simulink model "ADCSSimulator"  (R2024a)
settings: Solver=ode4  StartTime=0.0  StopTime=600  FixedStep=0.01  MaxStep=0.1  RelTol=1e-3  AbsTol=1e-3
values from neighbouring files (symbols this model uses):
  ActuatorAllocationMatrix = ActuatorPhysicalMatrix' * inv(ActuatorPhysicalMatrix * ActuatorPhysicalMatrix')    [set_Init.m]
  ActuatorPhysicalMatrix = [1, 0, 0, 0 ... (first row only)    [set_Init.m]
  albedo_irradiance = 300    [set_Init.m]
  b = 0    [set_Init.m]
  Cd = 2.2    [set_Init.m]
  h_bias = [0; 0; 0]    [set_Init.m]
  J = 4.0e-3 / 628    (= 6.36942675159e-06)    [set_Init.m]
  k_Bdot = ((4 * pi * 0.5236 * 0.0055) / (5677.2 * (4.5e-5)^2))    (= 3147.8423197)    [set_Init.m]
  K_E = K_T    (= 0.0022)    [set_Init.m]
  K_T = 0.0022    [set_Init.m]
  P0 = blkdiag(P0_att, P0_bias)    [set_Init.m]
  P0_att = eye(3) * initial_variance_rad2    [set_Init.m]
  PowerVoltageBus_01 = 3.3    [set_Init.m]
  PowerVoltageBus_02 = 3.3    [set_Init.m]
  PowerVoltageBus_03 = 3.3    [set_Init.m]
  PowerVoltageBus_04 = 3.3    [set_Init.m]
  PowerVoltageBus_05 = 3.3    [set_Init.m]
  PowerVoltageBus_06 = 3.3    [set_Init.m]
  PowerVoltageBus_07 = 3.3    [set_Init.m]
  PowerVoltageBus_08 = 3.3    [set_Init.m]
  PowerVoltageBus_09 = 3.3    [set_Init.m]
  PowerVoltageBus_10 = 3.3    [set_Init.m]
  PowerVoltageBus_11 = 3.3    [set_Init.m]
  PowerVoltageBus_12 = 0.0    (= 0)    [set_Init.m]
  PowerVoltageBus_13 = 0.0    (= 0)    [set_Init.m]
  PowerVoltageBus_14 = 0.0    (= 0)    [set_Init.m]
  PowerVoltageBus_15 = 0.0    (= 0)    [set_Init.m]
  R = 2.0    (= 2)    [set_Init.m]
  ressidual_m = [3e-4; -2e-4; 1e-4]    [set_Init.m]
  solar_irradiance = 1361    [set_Init.m]
  surface_areas = [A_xy, A_yz, A_xz, A_xy, A_yz, A_xz]    [set_Init.m]
  surface_normals_body = [eye(3) -eye(3)]    [set_Init.m]
  surface_positions_body = [       hx,   0,   0 ... (first row only)    [set_Init.m]
  surface_reflectivities = [0.9 0.8 0.9 0.9 0.9 0.9]    [set_Init.m]
  Switch_01 = 1    [set_Init.m]
  Switch_02 = 1    [set_Init.m]
  Switch_03 = 1    [set_Init.m]
  Switch_04 = 1    [set_Init.m]
  Switch_05 = 1    [set_Init.m]
  Switch_06 = 1    [set_Init.m]
  Switch_07 = 1    [set_Init.m]
  Switch_08 = 1    [set_Init.m]
  Switch_09 = 1    [set_Init.m]
  Switch_10 = 1    [set_Init.m]
  Switch_11 = 1    [set_Init.m]
  Switch_12 = 0    [set_Init.m]
  Switch_13 = 0    [set_Init.m]
  Switch_14 = 0    [set_Init.m]
  Switch_15 = 0    [set_Init.m]
  visSampleTime = 0.1    [set_Init.m]
undefined symbols (not defined in the file or in its folder): attitude, Controller, epoch, IAU, juliandate, Kd, km, Kp, m, rad, s, satellite, SGP4_parameters, simulator, UKF_parameters, WMM2020
libraries: sharedtransform x27, aerolibutil x22, aerolibconvert2 x18, simulink_extras x16, matrix_library x6, aerolibtransform2 x4, vrlib x2, aerolibgravity2 x2, aerolibobsolete x1, aerolibattitudesys x1, simulink x1
(part 7 of 8)

== matlab function ADCSSimulator/ADCS/ADCS Software/Onboard Reference Frames Transformations Manager1/Ensure Quaternion Continuity1/Ensure Quaternion Continuity ==
  data: q_new input; q_out output; q_prev input
function q_out = quaternion_continuity(q_new, q_prev)
%%%%%%%%%%%%%%%%%%%%%%%%%%%%%%%%%%%%%%%%%%%%%%%%%%%%%%%%%%%%%%%%%%%%%%%%
%   QUATERNION_CONTINUITY Ensures continuous quaternion output.
%
%   q_out = ensure_quaternion_continuity(q_new, q_prev) selects between
%   q_new and -q_new to ensure the shortest rotational path from q_prev,
%   preventing sign-flipping discontinuities in simulations.
%
%   Inputs:
%       q_new   - 4x1 newly calculated quaternion. Can be in either
%                 scalar-first or scalar-last format.
%       q_prev  - 4x1 quaternion from the previous time step. Must be in
%                 the same format as q_new.
%
%   Output:
%       q_out   - The 4x1 quaternion (either q_new or -q_new) that is
%                 mathematically closer to q_prev.
%%%%%%%%%%%%%%%%%%%%%%%%%%%%%%%%%%%%%%%%%%%%%%%%%%%%%%%%%%%%%%%%%%%%%%%%

    % 1. Input Validation (optional for Simulink if types are enforced)
    % coder.extrinsic('error'); % Uncomment if you need error checking
    % if ~isequal(size(q_new), [4,1]) || ~isequal(size(q_prev), [4,1])
    %     error('Input quaternions must be 4x1 column vectors.');
    % end

    % 2. Calculate the Euclidean distance (norm) to both possible rotations
    % The quaternions q and -q represent the same physical rotation. We want
    % to choose the one that is numerically closer to the previous state to
    % avoid a "jump" in the data when plotted.
    dist_to_positive_q = norm(q_new - q_prev);
    dist_to_negative_q = norm(-q_new - q_prev);

    % 3. Select the quaternion on the shortest path
    if dist_to_negative_q < dist_to_positive_q
        q_out = -q_new;
    else
        q_out = q_new;
    end
end

== matlab function ADCSSimulator/ADCS/ADCS Software/Onboard Reference Frames Transformations Manager1/Ensure Quaternion Continuity2/Ensure Quaternion Continuity ==
  data: q_new input; q_out output; q_prev input
function q_out = quaternion_continuity(q_new, q_prev)
%%%%%%%%%%%%%%%%%%%%%%%%%%%%%%%%%%%%%%%%%%%%%%%%%%%%%%%%%%%%%%%%%%%%%%%%
%   QUATERNION_CONTINUITY Ensures continuous quaternion output.
%
%   q_out = ensure_quaternion_continuity(q_new, q_prev) selects between
%   q_new and -q_new to ensure the shortest rotational path from q_prev,
%   preventing sign-flipping discontinuities in simulations.
%
%   Inputs:
%       q_new   - 4x1 newly calculated quaternion. Can be in either
%                 scalar-first or scalar-last format.
%       q_prev  - 4x1 quaternion from the previous time step. Must be in
%                 the same format as q_new.
%
%   Output:
%       q_out   - The 4x1 quaternion (either q_new or -q_new) that is
%                 mathematically closer to q_prev.
%%%%%%%%%%%%%%%%%%%%%%%%%%%%%%%%%%%%%%%%%%%%%%%%%%%%%%%%%%%%%%%%%%%%%%%%

    % 1. Input Validation (optional for Simulink if types are enforced)
    % coder.extrinsic('error'); % Uncomment if you need error checking
    % if ~isequal(size(q_new), [4,1]) || ~isequal(size(q_prev), [4,1])
    %     error('Input quaternions must be 4x1 column vectors.');
    % end

    % 2. Calculate the Euclidean distance (norm) to both possible rotations
    % The quaternions q and -q represent the same physical rotation. We want
    % to choose the one that is numerically closer to the previous state to
    % avoid a "jump" in the data when plotted.
    dist_to_positive_q = norm(q_new - q_prev);
    dist_to_negative_q = norm(-q_new - q_prev);

    % 3. Select the quaternion on the shortest path
    if dist_to_negative_q < dist_to_positive_q
        q_out = -q_new;
    else
        q_out = q_new;
    end
end

== matlab function ADCSSimulator/ADCS/ADCS Software/Onboard Reference Frames Transformations Manager1/Ensure Quaternion Continuity3/Ensure Quaternion Continuity ==
  data: q_new input; q_out output; q_prev input
function q_out = quaternion_continuity(q_new, q_prev)
%%%%%%%%%%%%%%%%%%%%%%%%%%%%%%%%%%%%%%%%%%%%%%%%%%%%%%%%%%%%%%%%%%%%%%%%
%   QUATERNION_CONTINUITY Ensures continuous quaternion output.
%
%   q_out = ensure_quaternion_continuity(q_new, q_prev) selects between
%   q_new and -q_new to ensure the shortest rotational path from q_prev,
%   preventing sign-flipping discontinuities in simulations.
%
%   Inputs:
%       q_new   - 4x1 newly calculated quaternion. Can be in either
%                 scalar-first or scalar-last format.
%       q_prev  - 4x1 quaternion from the previous time step. Must be in
%                 the same format as q_new.
%
%   Output:
%       q_out   - The 4x1 quaternion (either q_new or -q_new) that is
%                 mathematically closer to q_prev.
%%%%%%%%%%%%%%%%%%%%%%%%%%%%%%%%%%%%%%%%%%%%%%%%%%%%%%%%%%%%%%%%%%%%%%%%

    % 1. Input Validation (optional for Simulink if types are enforced)
    % coder.extrinsic('error'); % Uncomment if you need error checking
    % if ~isequal(size(q_new), [4,1]) || ~isequal(size(q_prev), [4,1])
    %     error('Input quaternions must be 4x1 column vectors.');
    % end

    % 2. Calculate the Euclidean distance (norm) to both possible rotations
    % The quaternions q and -q represent the same physical rotation. We want
    % to choose the one that is numerically closer to the previous state to
    % avoid a "jump" in the data when plotted.
    dist_to_positive_q = norm(q_new - q_prev);
    dist_to_negative_q = norm(-q_new - q_prev);

    % 3. Select the quaternion on the shortest path
    if dist_to_negative_q < dist_to_positive_q
        q_out = -q_new;
    else
        q_out = q_new;
    end
end

== matlab function ADCSSimulator/ADCS/ADCS Software/Onboard Reference Frames Transformations Manager1/Ensure Quaternion Continuity4/Ensure Quaternion Continuity ==
  data: q_new input; q_out output; q_prev input
function q_out = quaternion_continuity(q_new, q_prev)
%%%%%%%%%%%%%%%%%%%%%%%%%%%%%%%%%%%%%%%%%%%%%%%%%%%%%%%%%%%%%%%%%%%%%%%%
%   QUATERNION_CONTINUITY Ensures continuous quaternion output.
%
%   q_out = ensure_quaternion_continuity(q_new, q_prev) selects between
%   q_new and -q_new to ensure the shortest rotational path from q_prev,
%   preventing sign-flipping discontinuities in simulations.
%
%   Inputs:
%       q_new   - 4x1 newly calculated quaternion. Can be in either
%                 scalar-first or scalar-last format.
%       q_prev  - 4x1 quaternion from the previous time step. Must be in
%                 the same format as q_new.
%
%   Output:
%       q_out   - The 4x1 quaternion (either q_new or -q_new) that is
%                 mathematically closer to q_prev.
%%%%%%%%%%%%%%%%%%%%%%%%%%%%%%%%%%%%%%%%%%%%%%%%%%%%%%%%%%%%%%%%%%%%%%%%

    % 1. Input Validation (optional for Simulink if types are enforced)
    % coder.extrinsic('error'); % Uncomment if you need error checking
    % if ~isequal(size(q_new), [4,1]) || ~isequal(size(q_prev), [4,1])
    %     error('Input quaternions must be 4x1 column vectors.');
    % end

    % 2. Calculate the Euclidean distance (norm) to both possible rotations
    % The quaternions q and -q represent the same physical rotation. We want
    % to choose the one that is numerically closer to the previous state to
    % avoid a "jump" in the data when plotted.
    dist_to_positive_q = norm(q_new - q_prev);
    dist_to_negative_q = norm(-q_new - q_prev);

    % 3. Select the quaternion on the shortest path
    if dist_to_negative_q < dist_to_positive_q
        q_out = -q_new;
    else
        q_out = q_new;
    end
end

== matlab function ADCSSimulator/ADCS/ADCS Software/Onboard Reference Frames Transformations Manager1/Ensure Quaternion Continuity5/Ensure Quaternion Continuity ==
  data: q_new input; q_out output; q_prev input
function q_out = quaternion_continuity(q_new, q_prev)
%%%%%%%%%%%%%%%%%%%%%%%%%%%%%%%%%%%%%%%%%%%%%%%%%%%%%%%%%%%%%%%%%%%%%%%%
%   QUATERNION_CONTINUITY Ensures continuous quaternion output.
%
%   q_out = ensure_quaternion_continuity(q_new, q_prev) selects between
%   q_new and -q_new to ensure the shortest rotational path from q_prev,
%   preventing sign-flipping discontinuities in simulations.
%
%   Inputs:
%       q_new   - 4x1 newly calculated quaternion. Can be in either
%                 scalar-first or scalar-last format.
%       q_prev  - 4x1 quaternion from the previous time step. Must be in
%                 the same format as q_new.
%
%   Output:
%       q_out   - The 4x1 quaternion (either q_new or -q_new) that is
%                 mathematically closer to q_prev.
%%%%%%%%%%%%%%%%%%%%%%%%%%%%%%%%%%%%%%%%%%%%%%%%%%%%%%%%%%%%%%%%%%%%%%%%

    % 1. Input Validation (optional for Simulink if types are enforced)
    % coder.extrinsic('error'); % Uncomment if you need error checking
    % if ~isequal(size(q_new), [4,1]) || ~isequal(size(q_prev), [4,1])
    %     error('Input quaternions must be 4x1 column vectors.');
    % end

    % 2. Calculate the Euclidean distance (norm) to both possible rotations
    % The quaternions q and -q represent the same physical rotation. We want
    % to choose the one that is numerically closer to the previous state to
    % avoid a "jump" in the data when plotted.
    dist_to_positive_q = norm(q_new - q_prev);
    dist_to_negative_q = norm(-q_new - q_prev);

    % 3. Select the quaternion on the shortest path
    if dist_to_negative_q < dist_to_positive_q
        q_out = -q_new;
    else
        q_out = q_new;
    end
end

== matlab function ADCSSimulator/ADCS/ADCS Software/Onboard Reference Frames Transformations Manager1/MATLAB Function ==
  data: r input; SemiMajorAxis output; v input; mu input; Eccentricity output; Inclination output; RightAscension output; ArgumentOfPerigee output; TrueAnomaly output; TrueLongitude output; ArgumentOfLatitude output; LongitudeOfPeriapsis output; SemilatusRectum output; OrbOmega output
%----------------------- Begin Code Sequence -----------------------------%
% Purpose:                                                                %
% Convert a given set of state vectors in ECI reference frame to orbital  %
% elements.                                                               %
%-------------------------------------------------------------------------%
%                                                                         %
% Inputs:                                                                 %
%--------                                                                  
%r_ECI                  [3 x N]                         Position Vector in
%                                                       ECI coordinate
%                                                       frame of reference
%
%v_ECI                  [3 x N]                         Velocity vector in
%                                                       ECI coordinate
%                                                       frame of reference
%
%mu                     double                          Gravitational Constant
%                                                       Defaults to Earth if
%                                                       not specified
% Outputs:
%---------                                                                %
%a                      [1 x N]                         Semi-Major Axis
%                                                       (m)
%
%eMag                   [1 x N]                         Eccentricity
%                                                       (unitless)
%
%i                      [1 x N]                         inclination
%                                                       (rad)
%
%O                      [1 x N]                         Right Ascention of
%                                                       the ascending node
%                                                       (rad)
%
%o                      [1 x N]                         Argument of perigee
%                                                       (rad)
%
%M                      [1 x N]                         Mean Anomaly
%                                                       (rad)
%
%truLon                 [1 x N]                         True Longitude
%                                                       (rad)
%
%argLat                 [1 x N]                         Argument of Latitude
%                                                       (rad)
%
%lonPer                 [1 x N]                         Longitude of Periapse
%                                                       (rad)
%
%p                      [1 x N]                         Semilatus Rectum
%                                                       (m)
%
%OrbOmega                                               Orbital Frame
%                                                       angular velocity
%                                                       (rad)
% References:
%-------------
%Vallado,D. Fundamentals of Astrodynamics and Applications. 2007.
%
% Function Dependencies:
%------------------
%None
%------------------------------------------------------------------       %
% Programed by Darin Koblick  03-04-2012                                  %
% modified by A.H.Khodabakhsh 10-01-2021                                  %
% Updated to address circular equatorial orbits       12/12/2013          %
%------------------------------------------------------------------       %
function [SemiMajorAxis,Eccentricity,Inclination,RightAscension,ArgumentOfPerigee,TrueAnomaly,...
          TrueLongitude,ArgumentOfLatitude,LongitudeOfPeriapsis,SemilatusRectum,OrbOmega] = ...
          StateVector2KeplerianOrbitalElemets(r,v,mu)
% if ~exist('mu','var');  t = getConst(); mu = t.Earth.Mu; end
%Specific angular momentum
h = cross(r,v);
n = cross(repmat([0;0;1],[1,size(r,2)]),h); nMag = sqrt(sum(n.^2,1));
vMag = sqrt(sum(v.^2,1)); 
rMag = sqrt(sum(r.^2,1)); 
hMag = sqrt(sum(h.^2,1));
e = (1./mu).*(bsxfun(@times,(vMag.^2 - mu./rMag),r) - bsxfun(@times,dot(r,v),v)); 
Eccentricity = sqrt(sum(e.^2,1));
zeta = (vMag.^2)./2 - mu./rMag;
%Special Procedure when we have a parabolic orbit
idx = Eccentricity ~= 1;
SemiMajorAxis = zeros(size(Eccentricity));
SemilatusRectum = zeros(size(Eccentricity));
if any(idx)
    SemiMajorAxis(idx) = -mu./(2.*zeta(idx)); 
    SemilatusRectum(idx) = SemiMajorAxis(idx).*(1-Eccentricity(idx).^2); 
else
    SemiMajorAxis(idx) = Inf; 
    SemilatusRectum(idx) = (hMag(idx).^2)./mu; 
end
%Compute the angles
Inclination             = acos(double(single(   h(3,:)./hMag)                   )); 
RightAscension          = acos(double(single(   n(1,:)./nMag)                   ));
ArgumentOfPerigee       = acos(double(single(   dot(n,e)./(nMag.*Eccentricity)) ));
TrueAnomaly             = acos(double(single(   dot(e,r)./(Eccentricity.*rMag)) ));
LongitudeOfPeriapsis    = acos(double(single(   e(1,:)./Eccentricity)           ));
ArgumentOfLatitude      = acos(double(single(   dot(n,r)./(nMag.*rMag))         ));
TrueLongitude           = acos(double(single(   r(1,:)./rMag)                   ));
%Account for those cases where satellite is in circular orbit
         RightAscension   (  n(1,:) == 0) = 0;
       ArgumentOfPerigee  (dot(n,e) == 0) = 0;
      LongitudeOfPeriapsis(  e(1,:) == 0) = 0;
          TrueAnomaly     (dot(e,r) == 0) = 0;
       ArgumentOfLatitude (dot(n,r) == 0) = 0;
%Apply Quadrant Checks to All Determined Angles
idx = n(2,:) < 0; if any(idx),  RightAscension(idx) = 2*pi - RightAscension(idx);  end;
idx = e(3,:) < 0; if any(idx), ArgumentOfPerigee(idx) = 2*pi - ArgumentOfPerigee(idx); end;
idx = dot(r,v) < 0; if any(idx), TrueAnomaly(idx) = 2*pi - TrueAnomaly(idx); end;
idx = e(2,:) < 0; if any(idx), LongitudeOfPeriapsis(idx) = 2*pi-LongitudeOfPeriapsis(idx);  end;
idx = r(3,:) < 0; if any(idx), ArgumentOfLatitude(idx) = 2*pi - ArgumentOfLatitude(idx); end;
idx = r(2,:) < 0; if any(idx), TrueLongitude(idx) = 2*pi - TrueLongitude(idx); end;

rv = zeros(3,1);
rv(:)=cross(r,v); norm_r = norm(r);
OrbOmega = [0;
            dot(v,cross(r./norm_r,rv./norm(rv)))/norm_r;
            0];

% % convert radians to degrees
% r2d = @(x) x.*(180./pi);
% Inclination          = r2d(Inclination         );
% RightAscension       = r2d(RightAscension      );
% ArgumentOfPerigee    = r2d(ArgumentOfPerigee   );
% TrueAnomaly          = r2d(TrueAnomaly         );
% TrueLongitude        = r2d(TrueLongitude       );
% ArgumentOfLatitude   = r2d(ArgumentOfLatitude  );
% LongitudeOfPeriapsis = r2d(LongitudeOfPeriapsis);
% OrbOmega             = r2d(OrbOmega            );
end

== matlab function ADCSSimulator/ADCS/ADCS Software/Attitude Determination/Attitude Estimation Algorithm (MEKF)/Ensure Quaternion Continuity/Ensure Quaternion Continuity ==
  data: q_new input; q_out output; q_prev input
function q_out = quaternion_continuity(q_new, q_prev)
%%%%%%%%%%%%%%%%%%%%%%%%%%%%%%%%%%%%%%%%%%%%%%%%%%%%%%%%%%%%%%%%%%%%%%%%
%   QUATERNION_CONTINUITY Ensures continuous quaternion output.
%
%   q_out = ensure_quaternion_continuity(q_new, q_prev) selects between
%   q_new and -q_new to ensure the shortest rotational path from q_prev,
%   preventing sign-flipping discontinuities in simulations.
%
%   Inputs:
%       q_new   - 4x1 newly calculated quaternion. Can be in either
%                 scalar-first or scalar-last format.
%       q_prev  - 4x1 quaternion from the previous time step. Must be in
%                 the same format as q_new.
%
%   Output:
%       q_out   - The 4x1 quaternion (either q_new or -q_new) that is
%                 mathematically closer to q_prev.
%%%%%%%%%%%%%%%%%%%%%%%%%%%%%%%%%%%%%%%%%%%%%%%%%%%%%%%%%%%%%%%%%%%%%%%%

    % 1. Input Validation (optional for Simulink if types are enforced)
    % coder.extrinsic('error'); % Uncomment if you need error checking
    % if ~isequal(size(q_new), [4,1]) || ~isequal(size(q_prev), [4,1])
    %     error('Input quaternions must be 4x1 column vectors.');
    % end

    % 2. Calculate the Euclidean distance (norm) to both possible rotations
    % The quaternions q and -q represent the same physical rotation. We want
    % to choose the one that is numerically closer to the previous state to
    % avoid a "jump" in the data when plotted.
    dist_to_positive_q = norm(q_new - q_prev);
    dist_to_negative_q = norm(-q_new - q_prev);

    % 3. Select the quaternion on the shortest path
    if dist_to_negative_q < dist_to_positive_q
        q_out = -q_new;
    else
        q_out = q_new;
    end
end

== matlab function ADCSSimulator/ADCS/ADCS Software/Attitude Determination/Attitude Estimation Algorithm (MEKF)/MATLAB Function ==
  data: q_est output; b_est output; P_est output; q_feedback input; b_feedback input; P_feedback input; gyro_meas input; b_sun input; b_mag input; r_sun input; r_mag input; dt input; Q_v input; Q_u input; R_sun input; R_mag input; time input; q_quest input
function [q_est, b_est, P_est] = mekf_quest_reset( ...
    q_feedback, b_feedback, P_feedback, ...
    gyro_meas, b_sun, b_mag, r_sun, r_mag, ...
    dt, Q_v, Q_u, R_sun, R_mag, ...
    time, q_quest)
% MEKF_QUEST_RESET (6-State, Batch Update, One-Time Init)
%
% This function implements a 6-state MEKF with a one-time state reset
% using an external QUEST solution at a specified time.
%
% QUATERNION CONVENTION
% This function uses the standard Hamilton convention: q = [w; x; y; z].

% =========================================================================
% 0) INITIALIZATION & STATE MANAGEMENT
% =========================================================================
QUEST_INIT_TIME = 3.0; % The time to perform the reset

if isempty(P_feedback) || norm(P_feedback) == 0
    q_minus = [1; 0; 0; 0];
    b_minus = [0; 0; 0];
    P_att_initial = eye(3) * (pi^2);
    P_bias_initial = eye(3) * (1e-4);
    P_minus = blkdiag(P_att_initial, P_bias_initial);
else
    q_minus = q_feedback;
    b_minus = b_feedback;
    P_minus = P_feedback;
end

% --- One-Time QUEST Initialization ---
if abs(time - QUEST_INIT_TIME) < (dt / 2) && ~any(isnan(q_quest))
    % ACTION: Overwrite attitude with the QUEST solution
    q_minus = q_quest;
    
    % ACTION: Create a new covariance matrix for the attitude part
    % This is a tuning parameter: our assumed uncertainty after a QUEST reset.
    QUEST_RESET_STD_DEV_DEG = 1.0; % e.g., Assume QUEST is accurate to 1 degree
    QUEST_RESET_STD_DEV_RAD = QUEST_RESET_STD_DEV_DEG * (pi/180);
    P_att_after_quest = eye(3) * QUEST_RESET_STD_DEV_RAD^2;
    
    % Keep the filter's current estimate of the bias covariance
    P_bias_current = P_minus(4:6, 4:6);
    
    % Combine to form the new 6x6 covariance
    P_minus = blkdiag(P_att_after_quest, P_bias_current);
end
q_minus = q_minus / norm(q_minus);

% =========================================================================
% 1) PREDICTION (PROPAGATION)
% =========================================================================
omega = gyro_meas - b_minus;

theta_vec = omega * dt;
phi = norm(theta_vec);
if phi > 1e-9
    axis = theta_vec / phi;
    q_delta = [cos(phi / 2); sin(phi / 2) * axis];
else
    q_delta = [1; 0; 0; 0];
end
q_propagated = quat_mult(q_minus, q_delta);
q_propagated = q_propagated / norm(q_propagated);

skew_omega = cross_matrix(omega);
F = [-skew_omega, -eye(3); zeros(3,3), zeros(3,3)];
Phi = expm(F * dt);
Qd = blkdiag(Q_v, Q_u) * dt;
P_propagated = Phi * P_minus * Phi' + Qd;
P_propagated = 0.5 * (P_propagated + P_propagated');

% =========================================================================
% 2) BATCH MEASUREMENT UPDATE (ROBUST PRE-ALLOCATION VERSION)
% =========================================================================
q_est = q_propagated;
b_est = b_minus;
P_est = P_propagated;

is_sun_available = ~any(isnan(b_sun));
is_mag_available = ~any(isnan(b_mag));

% Proceed only if there is at least one valid measurement
if is_sun_available || is_mag_available
    A = quat_to_dcm(q_propagated);

    % 1. Determine size and pre-allocate matrices
    if is_sun_available && is_mag_available
        meas_size = 6;
    else
        meas_size = 3;
    end
    z = zeros(meas_size, 1);
    h = zeros(meas_size, 1);
    H = zeros(meas_size, 6);
    R = zeros(meas_size, meas_size);
    
    % 2. Fill the matrices based on available sensors
    if is_sun_available && is_mag_available
        % Case 1: Both sensors
        z = [b_sun; b_mag];
        h_sun = A * r_sun;
        h_mag = A * r_mag;
        h = [h_sun; h_mag];
        H_sun = [cross_matrix(h_sun), zeros(3,3)];
        H_mag = [cross_matrix(h_mag), zeros(3,3)];
        H = [H_sun; H_mag];
        R = blkdiag(R_sun, R_mag);
        
    elseif is_sun_available % Case 2: Sun only
        z = b_sun;
        h = A * r_sun;
        H = [cross_matrix(h), zeros(3,3)];
        R = R_sun;

    else % Case 3: Mag only (is_mag_available must be true)
        z = b_mag;
        h = A * r_mag;
        H = [cross_matrix(h), zeros(3,3)];
        R = R_mag;
    end
    
    % 3. Perform the Kalman Update
    % This code now runs safely with guaranteed, fully-defined matrices.
    y = z - h;
    S = H * P_propagated * H' + R;
    K = (P_propagated * H') / S;
    
    delta_x = K * y;
    delta_a = delta_x(1:3);
    delta_b = delta_x(4:6);

    delta_q = [1; 0.5 * delta_a];
    delta_q = delta_q / norm(delta_q);
    
    q_est = quat_mult(q_propagated, delta_q);
    b_est = b_minus + delta_b;

    IKH = eye(6) - K * H;
    P_est = IKH * P_propagated * IKH' + K*R*K';
    P_est = 0.5 * (P_est + P_est');
end

% =========================================================================
% HELPER FUNCTIONS
% =========================================================================
function C = cross_matrix(v)
    C = [  0   -v(3)  v(2); v(3)   0   -v(1); -v(2)  v(1)   0  ];
end

function r = quat_mult(q1, q2)
    w1 = q1(1); v1 = q1(2:4);
    w2 = q2(1); v2 = q2(2:4);
    w = w1*w2 - dot(v1, v2);
    v = w1*v2 + w2*v1 + cross(v1, v2);
    r = [w; v];
end

function A = quat_to_dcm(q)
    w = q(1); v = q(2:4);
    skew_v = cross_matrix(v);
    A = eye(3) + 2*w*skew_v + 2*skew_v*skew_v;
end
end

== matlab function ADCSSimulator/ADCS/ADCS Software/Attitude Determination/Static Attitude Determination Algorithm (QUEST)/Ensure Quaternion Continuity1/Ensure Quaternion Continuity ==
  data: q_new input; q_out output; q_prev input
function q_out = quaternion_continuity(q_new, q_prev)
%%%%%%%%%%%%%%%%%%%%%%%%%%%%%%%%%%%%%%%%%%%%%%%%%%%%%%%%%%%%%%%%%%%%%%%%
%   QUATERNION_CONTINUITY Ensures continuous quaternion output.
%
%   q_out = ensure_quaternion_continuity(q_new, q_prev) selects between
%   q_new and -q_new to ensure the shortest rotational path from q_prev,
%   preventing sign-flipping discontinuities in simulations.
%
%   Inputs:
%       q_new   - 4x1 newly calculated quaternion. Can be in either
%                 scalar-first or scalar-last format.
%       q_prev  - 4x1 quaternion from the previous time step. Must be in
%                 the same format as q_new.
%
%   Output:
%       q_out   - The 4x1 quaternion (either q_new or -q_new) that is
%                 mathematically closer to q_prev.
%%%%%%%%%%%%%%%%%%%%%%%%%%%%%%%%%%%%%%%%%%%%%%%%%%%%%%%%%%%%%%%%%%%%%%%%

    % 1. Input Validation (optional for Simulink if types are enforced)
    % coder.extrinsic('error'); % Uncomment if you need error checking
    % if ~isequal(size(q_new), [4,1]) || ~isequal(size(q_prev), [4,1])
    %     error('Input quaternions must be 4x1 column vectors.');
    % end

    % 2. Calculate the Euclidean distance (norm) to both possible rotations
    % The quaternions q and -q represent the same physical rotation. We want
    % to choose the one that is numerically closer to the previous state to
    % avoid a "jump" in the data when plotted.
    dist_to_positive_q = norm(q_new - q_prev);
    dist_to_negative_q = norm(-q_new - q_prev);

    % 3. Select the quaternion on the shortest path
    if dist_to_negative_q < dist_to_positive_q
        q_out = -q_new;
    else
        q_out = q_new;
    end
end

== matlab function ADCSSimulator/ADCS/ADCS Software/Attitude Determination/Static Attitude Determination Algorithm (QUEST)/Static Attitude Determination Algorithm (QUEST) ==
  data: r_sun input; q output; P output; r_mag input; b_sun input; b_mag input; w_sun input; w_mag input; q_prev input; lambda_max output
function [q, P, lambda_max] = quest_algorithm(r_sun, r_mag, b_sun, b_mag, w_sun, w_mag, q_prev)
%%%%%%%%%%%%%%%%%%%%%%%%%%%%%%%%%%%%%%%%%%%%%%%%%%%%%%%%%%%%%%%%%%%%%%%%%%%%%%%%%%%%%%%%%%%%%%%
% QUEST_ALGORITHM Estimates attitude quaternion and its covariance using QUEST.
%
%   This function is robust to sensor outages and poor geometric
%    conditions (collinear vectors). It does NOT perform continuity checks;
%    that should be handled at the system level after this function's output.
%
%   Inputs:
%       r_sun   - 3x1 Sun vector in the reference (ICRF) frame.
%       r_mag   - 3x1 Magnetic field vector in the reference (ICRF) frame.
%       b_sun   - 3x1 Sun vector measured in the body frame. Can be NaN.
%       b_mag   - 3x1 Magnetic field vector measured in the body frame. Can be NaN.
%       w_sun   - Scalar weight for the Sun vector measurement.
%       w_mag   - Scalar weight for the Magnetic field measurement.
%       q_prev  - 4x1 quaternion from the previous time step, assumed to be
%                 in [scalar, vector] format. Used for graceful failure.
%
%   Outputs:
%       q          - 4x1 attitude quaternion in [scalar, vector] format.
%       P          - 3x3 attitude error covariance matrix. -> ** this matrix
%       is an approximated matrix**
%       lambda_max - The maximum eigenvalue of the K matrix.
%%%%%%%%%%%%%%%%%%%%%%%%%%%%%%%%%%%%%%%%%%%%%%%%%%%%%%%%%%%%%%%%%%%%%%%%%%%%%%%%%%%%%%%%%%%%%%%

    % ** Pre-allocate outputs to satisfy Simulink's fixed-size requirement
    q = zeros(4, 1);
    P = eye(3) * 1e6; % Default high uncertainty
    lambda_max = 0.0;

    % ** Sanitize Inputs and Determine Validity
    vectors = struct('r', {r_sun, r_mag}, ...
                     'b', {b_sun, b_mag}, ...
                     'w', {w_sun, w_mag}, ...
                     'valid', {false, false});
    
    for i = 1:2
        if ~any(isnan(vectors(i).b)) && ~any(isinf(vectors(i).b)) && ...
           norm(vectors(i).r) > eps && norm(vectors(i).b) > eps
            
            vectors(i).valid = true;
            vectors(i).r = vectors(i).r / norm(vectors(i).r);
            vectors(i).b = vectors(i).b / norm(vectors(i).b);
        end
    end

    % ** Filter for Valid Measurements
    valid_indices = [vectors.valid];
    if ~any(valid_indices)
        q = q_prev;
        return;
    end
    
    b_valid = [vectors(valid_indices).b];
    r_valid = [vectors(valid_indices).r];
    w_valid_row = [vectors(valid_indices).w];
    
    % *** Robustness Fix: Force w_valid to be a column vector to ensure its
    %  dimensions are unambiguous for the Coder when its size changes.
    w_valid = w_valid_row(:);
    
    w_valid = w_valid / sum(w_valid, 'all');

    % ** Robustness Check for Collinearity
    if size(b_valid, 2) == 2
        dot_product = abs(dot(b_valid(:,1), b_valid(:,2)));
        if dot_product > 0.999
            if w_valid(1) < w_valid(2)
                b_valid = b_valid(:,2);
                r_valid = r_valid(:,2);
                w_valid = 1;
            else
                b_valid = b_valid(:,1);
                r_valid = r_valid(:,1);
                w_valid = 1;
            end
        end
    end
    
    % 1. Construct the Attitude Profile Matrix (B)
    B = b_valid * diag(w_valid) * r_valid';

    % 2. Form the K matrix
    S = B + B';
    sigma = trace(B);
    Z = [B(2,3) - B(3,2); B(3,1) - B(1,3); B(1,2) - B(2,1)];
    K = [S - sigma * eye(3), Z; Z', sigma];

    % 3. Find eigenvector and eigenvalue
    [V, D] = eig(K, 'vector');
    [max_eigenvalue, max_idx] = max(real(D));
    q_new_internal = real(V(:, max_idx));
    lambda_max = max_eigenvalue;

    % 4. Calculate Attitude Error Covariance Matrix (P)
    information_matrix = sigma * eye(3) - S;
    if rcond(information_matrix) < eps
        P = pinv(information_matrix);
    else
        P = inv(information_matrix);
    end
    
    % 5. Final Normalization & Format Conversion
    norm_q = norm(q_new_internal);
    if norm_q < eps
        q = q_prev;
        P = eye(3) * 1e6;
        lambda_max = 0.0;
    else
        q_normalized_internal = q_new_internal / norm_q;
        q = [q_normalized_internal(4); q_normalized_internal(1:3)];
    end
end

== matlab function ADCSSimulator/ADCS/ADCS Software/Attitude Guidance/MATLAB Function ==
  data: sI input; Sun_BodytoICRFQuaternions output; b_axis input
function Sun_BodytoICRFQuaternions = sunPointQuat(sI, b_axis)
% sI: 3×1 sun vector in inertial frame
% b_axis: 3×1 axis in body frame to point at the sun
% returns: quaternion q_des = [q0; qv]

  % rotation axis
  u = cross(b_axis, sI);
  if norm(u)<1e-8
    % already aligned or anti-aligned
    angle = acos(dot(b_axis, sI));
    if angle < 1e-6
      Sun_BodytoICRFQuaternions = [1;0;0;0];
      return
    else
      % 180° around any perpendicular axis
      u = null(b_axis.');
      u = u(:,1);
    end
  end

  angle = atan2(norm(u), dot(b_axis, sI));  
  u = u/norm(u);

  Sun_BodytoICRFQuaternions = [cos(angle/2);
           u*sin(angle/2)];
end

== matlab function ADCSSimulator/ADCS/ADCS Software/Orbit Detemination/Latching Logic/MATLAB Function4 ==
  data: r_eci_km input; x_initial output; v_eci_km_s input
function x_initial  = format_initial_state(r_eci_km, v_eci_km_s)
% format_initial_state Formats position and velocity into a state vector.
%
% Function Objective:
% This function serves as a simple utility to format the initial position
% and velocity vectors into the 6x1 state vector required by the Kalman filter.
%
% How to Use:
% In your Simulink model, take the position (r_ICRF) and velocity (v_ICRF)
% outputs from your main SGP4 propagator block at the first time step (t=0)
% and feed them into this function. The output will be the correctly
% formatted 'x_initial' vector needed to start the UKF.
%
% Inputs:
%   r_eci_km:   (3x1 double) The initial position vector from SGP4 [km].
%   v_eci_km_s: (3x1 double) The initial velocity vector from SGP4 [km/s].
%
% Output:
%   x_initial: (6x1 double) The initial state vector [r_eci_km; v_eci_km_s]
%                           formatted for the UKF.

    % --- Format the Output State Vector ---
    % The UKF expects a single 6x1 state vector, so we vertically stack
    % the 3x1 position vector on top of the 3x1 velocity vector.
    x_initial = [r_eci_km; v_eci_km_s];

end

== matlab function ADCSSimulator/ADCS/ADCS Software/Quaternion Error (deg) ==
  data: q_true input; error_angle_deg output; q_est input
function error_angle_deg = quaternion_angle_error(q_true, q_est)
% Calculates the angular error between two quaternions

% Inputs:
%   q_true: 4x1 true attitude quaternion [scalar; vector].
%   q_est:  4x1 estimated attitude quaternion [scalar; vector].
%
% Output:
%   error: 180-deg error.

    % Validate input dimensions.
    if ~isequal(size(q_true), [4,1]) || ~isequal(size(q_est), [4,1])
        error('Input quaternions must be 4x1 column vectors.');
    end

    % Step 1: Calculate the Error Quaternion
    % The error quaternion (delta_q) represents the rotation needed to get
    % from the estimated attitude to the true attitude.
    delta_q = quat_multiply(q_true, quat_inverse(q_est));

    % Step 2: Extract the Angular Error
    % The angle of rotation is calculated from the scalar part of the error
    % quaternion. The absolute value ensures we get the shortest path (<= 180 deg).
    scalar_part = abs(delta_q(1));
    
    % Clamp the value to 1.0 to prevent numerical errors from acos().
    scalar_part = min(1.0, scalar_part);
    
    error_angle_rad = 2 * acos(scalar_part);
    
    % Step 3: Convert to deg
    % Convert the angular error in degrees
    error_angle_deg = error_angle_rad * (180 / pi);
end

% Helper Functions for Quaternion Math
function q_out = quat_multiply(q1, q2)
    % Multiplies two quaternions, q1 * q2.
    s1 = q1(1); v1 = q1(2:4);
    s2 = q2(1); v2 = q2(2:4);
    
    s_out = s1*s2 - dot(v1, v2);
    v_out = s1*v2 + s2*v1 + cross(v1, v2);
    
    q_out = [s_out; v_out];
    % Re-normalize to prevent accumulation of floating-point errors.
    if norm(q_out) > 1e-9
        q_out = q_out / norm(q_out);
    else
        q_out = [1; 0; 0; 0]; % Return identity if result is zero
    end
end

function q_inv = quat_inverse(q)
    % The inverse of a unit quaternion is its conjugate.
    q_inv = [q(1); -q(2:4)];
end

== matlab function ADCSSimulator/ADCS/ADCS Software/Orbit Detemination/SGP4 Propagator ==
  data: epoch_julian_date_utc input; r_ICRF_km output; mean_motion_rad_per_min input; eccentricity input; inclination_rad input; raan_rad input; arg_of_perigee_rad input; v_ICRF_kms output; mean_anomaly_rad input; bstar_drag_term input; current_julian_date_utc input
function [r_ICRF_km, v_ICRF_kms] = propagate_from_tle(epoch_julian_date_utc, mean_motion_rad_per_min, eccentricity, inclination_rad, raan_rad, arg_of_perigee_rad, mean_anomaly_rad, bstar_drag_term, current_julian_date_utc)
% propagate_from_tle Propagates an orbit state from a TLE using SGP4.
%
% Function Objective:
% This function serves two critical roles in a robust ADCS:
%   1. Initialization: Provides the initial state vector [r, v] for a
%      high-fidelity estimator (like a UKF) when a new TLE is received.
%   2. Safe Mode Propagation: Acts as a stable, reliable, albeit lower-accuracy,
%      propagator if the primary estimator fails and the system enters a
%      safe mode.
%
% Inputs:
%   epoch_julian_date_utc:   (double) The reference epoch of the TLE [Julian Date, UTC].
%   mean_motion_rad_per_min: (double) The SGP4 mean motion [rad/min].
%   eccentricity:            (double) The eccentricity of the orbit [unitless].
%   inclination_rad:         (double) The orbital inclination [rad].
%   raan_rad:                (double) Right Ascension of the Ascending Node [rad].
%   arg_of_perigee_rad:      (double) Argument of Perigee [rad].
%   mean_anomaly_rad:        (double) The mean anomaly at epoch [rad].
%   bstar_drag_term:         (double) The B-star drag term [1/EarthRadii].
%   current_julian_date_utc: (double) The target time for state generation [Julian Date, UTC].
%
% Outputs:
%   r_ICRF_km:  (3x1 double) The propagated position vector in ICRF [km].
%   v_ICRF_kms: (3x1 double) The propagated velocity vector in ICRF [km/s].
%===============================================================================

    % --- Time Calculation ---
    tsince = (current_julian_date_utc - epoch_julian_date_utc) * 1440.0; % days to minutes

    % Section 1: Initialization and Mean Element Recovery
    xke = 0.07436691613317341; 
    j2 = 1.082616e-3;
    j3 = -2.53881e-6;
    j4 = -1.65597e-6;
    j3oj2 = j3 / j2;
    ae = 1.0;

    no_rev_per_day = mean_motion_rad_per_min * (1440.0 / (2.0 * pi));

    a1 = (xke / no_rev_per_day)^(2/3);
    cosio = cos(inclination_rad);
    theta2 = cosio^2;
    x3thm1 = 3.0 * theta2 - 1.0;
    betao2 = 1.0 - eccentricity^2;
    betao = sqrt(betao2);
    del1 = 1.5 * j2 * x3thm1 / (a1^2 * betao^3);
    ao = a1 * (1.0 - del1 * (0.5 + del1 * (1.0 + (134.0/81.0) * del1)));
    delo = 1.5 * j2 * x3thm1 / (ao^2 * betao^3);
    no_kozai = no_rev_per_day / (1.0 + delo);
    aodp = ao / (1.0 - delo);

    % Section 2: Secular Effects Calculation
    s4 = 78.0; 
    qoms24 = 1.8848033e-09; 
    perigee = (aodp * (1.0 - eccentricity) - ae) * 6378.135;
    
    if perigee < 156.0
        s4 = perigee - 78.0;
        if perigee < 98.0
            s4 = 20.0;
        end
        qoms24 = ((120.0 - s4) * ae / 6378.135)^4;
        s4 = s4 / 6378.135 + ae;
    end
    
    pinvsq = 1.0 / (aodp^2 * betao2^2);
    tsi = 1.0 / (aodp - s4);
    eta = aodp * eccentricity * tsi;
    etasq = eta^2;
    eeta = eccentricity * eta;
    psisq = abs(1.0 - etasq);
    coef = qoms24 * tsi^4;
    coef1 = coef / psisq^3.5;
    
    c2 = coef1 * no_kozai * (aodp * (1.0 + 1.5 * etasq + eeta * (4.0 + etasq)) + ...
        0.75 * j2 * tsi / psisq * x3thm1 * (8.0 + 24.0 * etasq + 3.0 * etasq^2));
    c1 = bstar_drag_term * c2;
    sinio = sin(inclination_rad);
    a3ovk2 = -j3oj2 * ae^3;
    c3 = coef * tsi^5 * a3ovk2 * no_kozai * ae * sinio / eccentricity;
    c4 = 2.0 * no_kozai * coef1 * aodp * betao2 * (eta * (2.0 + 0.5 * etasq) + ...
        eccentricity * (0.5 + 2.0 * etasq) - 2.0 * j2 * tsi / (aodp * psisq) * ...
        (-3.0 * x3thm1 * (1.0 - 2.0 * eeta + etasq * (1.5 - 0.5 * eeta)) + ...
        0.75 * (1.0 - theta2) * (2.0 * etasq - eeta * (1.0 + etasq)) * cos(2.0 * arg_of_perigee_rad)));
    c5 = 2.0 * coef1 * aodp * betao2 * (1.0 + 2.75 * (etasq + eeta) + eeta * etasq);
    
    theta4 = theta2^2;
    temp1 = 3.0 * j2 * pinvsq * no_kozai;
    temp2 = temp1 * j2 * pinvsq;
    temp3 = 1.25 * j4 * pinvsq * pinvsq * no_kozai;
    
    xmdot = no_kozai + 0.5 * temp1 * betao * x3thm1 + ...
        0.0625 * temp2 * betao * (13.0 - 78.0 * theta2 + 137.0 * theta4);
    xargpdot = -0.5 * temp1 * (1.0 - 5.0 * theta2) - ...
        0.0625 * temp2 * (7.0 - 114.0 * theta2 + 395.0 * theta4) + ...
        temp3 * (3.0 - 36.0 * theta2 + 49.0 * theta4);
    xnodot = -temp1 * cosio - 0.5 * temp2 * (4.0 - 19.0 * theta2) * cosio + ...
        2.0 * temp3 * (3.0 - 7.0 * theta2) * cosio;
        
    xmcof = -2.0/3.0 * coef * bstar_drag_term * ae / eeta;

    % Section 3: Propagation and Perturbation Application
    m_secular = mean_anomaly_rad + xmdot * tsince;
    argp_secular = arg_of_perigee_rad + xargpdot * tsince;
    node_secular = raan_rad + xnodot * tsince;
    
    ecc_secular = eccentricity;
    
    if c1 ~= 0.0
        delta_m = 1.0 + xmcof * tsince;
        m_secular = m_secular + bstar_drag_term * c2 * (tsince^2 / 4.0 + delta_m * tsince^3 / 12.0);
        argp_secular = argp_secular - c5 * (sin(m_secular) - sin(mean_anomaly_rad));
        node_secular = node_secular + c4 * (sin(m_secular) - sin(mean_anomaly_rad));
        delta_e = bstar_drag_term * c4 * (cos(m_secular) - cos(mean_anomaly_rad));
        ecc_secular = eccentricity - delta_e;
        if ecc_secular < 1e-6, ecc_secular = 1e-6; end
    end
    
    axn = ecc_secular * cos(argp_secular);
    ayn = ecc_secular * sin(argp_secular) - a3ovk2 * sinio;
    
    xl = mod(m_secular + argp_secular + node_secular, 2*pi);
    u = mod(xl - node_secular, 2*pi);
    eo1 = u;
    for i = 1:10
        e_new = eo1 + (u - ayn * cos(eo1) + axn * sin(eo1) - eo1) / ...
            (ayn * sin(eo1) + axn * cos(eo1) + 1.0);
        if abs(e_new - eo1) < 1e-12, break; end
        eo1 = e_new;
    end
    
    ecose = axn * cos(eo1) + ayn * sin(eo1);
    esine = axn * sin(eo1) - ayn * cos(eo1);
    
    n_secular = no_kozai + 1.5 * c1 * (tsince + 0.5 * bstar_drag_term * c2 * tsince^2);
    a_secular = (xke / n_secular)^(2/3);
    
    pl = a_secular * (1.0 - ecc_secular^2);
    r_osc = a_secular * (1.0 - ecose);
    rdot_osc = xke * sqrt(a_secular) * esine / r_osc;
    rvdot_osc = xke * sqrt(pl) / r_osc;
    
    beta = sqrt(1.0 - ecc_secular^2);
    temp = esine / (1.0 + beta);
    sinu = a_secular / r_osc * (sin(eo1) - ayn - axn * temp);
    cosu = a_secular / r_osc * (cos(eo1) - axn + ayn * temp);
    su = atan2(sinu, cosu);
    
    sin2u = 2.0 * sinu * cosu;
    cos2u = 2.0 * cosu^2 - 1.0;
    
    temp1 = 0.5 * j2 * (1.0 / pl)^2;
    temp2 = temp1 * (1.0 - 1.5 * theta2);
    
    delta_r = temp1 * (1.0 - theta2) * cos2u;
    delta_u = -0.25 * temp2 * (7.0 * theta2 - 1.0) * sin2u;
    delta_omega = 1.5 * temp2 * cosio * sin2u;
    delta_i = 1.5 * temp2 * cosio * sinio * cos2u;
    delta_rdot = -xke * temp1 * (1.0 - theta2) * sin2u * n_secular / sqrt(pl);
    delta_rvdot = xke * temp1 * ((1.0 - theta2) * cos2u + 1.5 * (1.0 - 1.5 * theta2)) * n_secular / sqrt(pl);
    
    r_osc = r_osc * (1.0 - 1.5 * temp2 * beta * x3thm1) + delta_r;
    u_osc = su + delta_u;
    omega_osc = node_secular + delta_omega;
    i_osc = inclination_rad + delta_i;
    rdot_osc = rdot_osc + delta_rdot;
    rvdot_osc = rvdot_osc + delta_rvdot;

    % Section 4: Final Position and Velocity Calculation
    sinu_osc = sin(u_osc); cosu_osc = cos(u_osc);
    sin_omega_osc = sin(omega_osc); cos_omega_osc = cos(omega_osc);
    sini_osc = sin(i_osc); cosi_osc = cos(i_osc);
    
    x = r_osc * (cosu_osc * cos_omega_osc - sinu_osc * sin_omega_osc * cosi_osc);
    y = r_osc * (cosu_osc * sin_omega_osc + sinu_osc * cos_omega_osc * cosi_osc);
    z = r_osc * (sinu_osc * sini_osc);
    
    vx = rdot_osc * x / r_osc + rvdot_osc * (-sinu_osc * cos_omega_osc - cosu_osc * sin_omega_osc * cosi_osc);
    vy = rdot_osc * y / r_osc + rvdot_osc * (-sinu_osc * sin_omega_osc + cosu_osc * cos_omega_osc * cosi_osc);
    vz = rdot_osc * z / r_osc + rvdot_osc * (cosu_osc * sini_osc);
    
    r_ICRF_km = [x; y; z] * 6378.135;
    v_ICRF_kms = [vx; vy; vz] * (6378.135 / 60.0);
end
